simulink model "NBMS_Fault"  (R2026b)
settings: Solver=FixedStepDiscrete  StopTime=25  FixedStep=0.1
settings Model: Creator=hp  LastModifiedBy=rathi
settings OptimizationCC: DefaultParameterBehavior=Inlined  DifferentSizesBufferReuse=on  EfficientTunableParamExpr=on  EnhancedBackFolding=on  OptimizationCustomize=off  OptimizeBlockOrder=speed  PassReuseOutputArgsAs=Individual arguments  RemoveInternalMemoryZeroInit=on  RemoveRootLevelIOMemoryZeroInit=on
settings DebuggingCC: ParameterTunabilityLossMsg=error
settings SFSimCC: MATLABDynamicMemAlloc=off
settings RTWCC: Description=Embedded Coder  GenCodeOnly=on  PackageGeneratedCodeAndArtifacts=on  SystemTargetFile=ert.tlc  TemplateMakefile=ert_default_tmf
settings CodeAppCC: ForceParamTrailComments=on  IgnoreCustomStorageClasses=off  InsertBlockDesc=on  OperatorAnnotations=on  SFDataObjDesc=on  SimulinkDataObjDesc=on
settings ERTTargetCC: DynamicArrayContainerType=coder::array  GenerateSampleERTMain=on
settings ConfigComp: DVDefectChecker=on  DVDetectOutOfBounds=on  DVHarnessSource=Signal Editor  DVModelReferenceHarness=on  DVTestSuiteOptimization=Auto

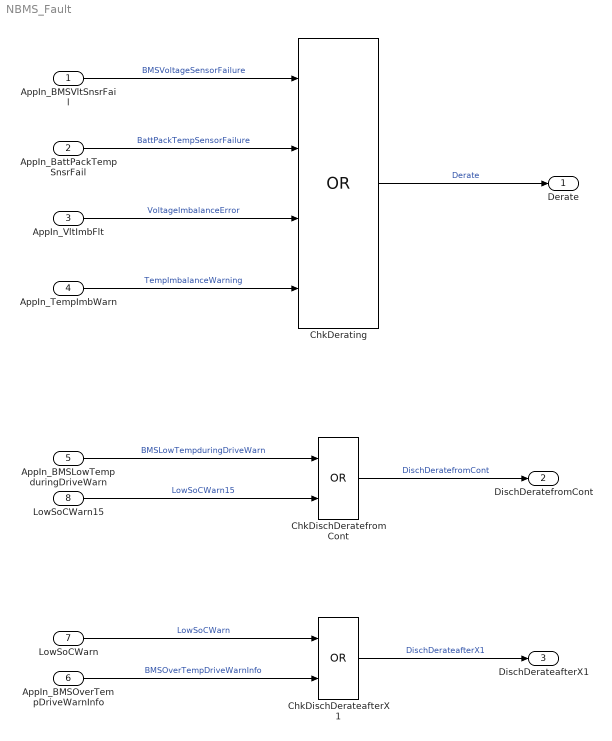
== system NBMS_Fault ==
  AppIn_BMSVltSnsrFail : Inport  OutDataTypeStr=boolean
  AppIn_BattPackTempSnsrFail : Inport  Port=2  OutDataTypeStr=boolean
  AppIn_VltImbFlt : Inport  Port=3  OutDataTypeStr=boolean
  AppIn_TempImbWarn : Inport  Port=4  OutDataTypeStr=boolean
  AppIn_BMSLowTempduringDriveWarn : Inport  Port=5  OutDataTypeStr=boolean
  AppIn_BMSOverTempDriveWarnInfo : Inport  Port=6  OutDataTypeStr=boolean
  LowSoCWarn : Inport  Port=7  OutDataTypeStr=boolean
  LowSoCWarn15 : Inport  Port=8  OutDataTypeStr=boolean
  ChkDerating : Logic  Operator=OR  Inputs=4  AllPortsSameDT=off  OutDataTypeStr=boolean
  ChkDischDerateafterX1 : Logic  Operator=OR  AllPortsSameDT=off  OutDataTypeStr=boolean
  ChkDischDeratefromCont : Logic  Operator=OR  AllPortsSameDT=off  OutDataTypeStr=boolean
  Derate : Outport
  DischDeratefromCont : Outport  Port=2  OutDataTypeStr=boolean
  DischDerateafterX1 : Outport  Port=3  OutDataTypeStr=boolean
  wires:
  AppIn_VltImbFlt/1 -> ChkDerating/3  "VoltageImbalanceError"
  AppIn_TempImbWarn/1 -> ChkDerating/4  "TempImbalanceWarning"
  AppIn_BattPackTempSnsrFail/1 -> ChkDerating/2  "BattPackTempSensorFailure"
  AppIn_BMSVltSnsrFail/1 -> ChkDerating/1  "BMSVoltageSensorFailure"
  ChkDerating/1 -> Derate/1  "Derate"
  AppIn_BMSLowTempduringDriveWarn/1 -> ChkDischDeratefromCont/1  "BMSLowTempduringDriveWarn"
  LowSoCWarn15/1 -> ChkDischDeratefromCont/2  "LowSoCWarn15"
  ChkDischDeratefromCont/1 -> DischDeratefromCont/1  "DischDeratefromCont"
  LowSoCWarn/1 -> ChkDischDerateafterX1/1  "LowSoCWarn"
  AppIn_BMSOverTempDriveWarnInfo/1 -> ChkDischDerateafterX1/2  "BMSOverTempDriveWarnInfo"
  ChkDischDerateafterX1/1 -> DischDerateafterX1/1  "DischDerateafterX1"
